simulink subsystem "UAV_model"  (R2025b)
settings: Solver=VariableStepAuto  StartTime=0.0  StopTime=10.0  RelTol=1e-3
values from neighbouring files (symbols this model uses):
  g_noise = 0.01    [random_init.m]
  Ts = 0.05    [generate_commande_preview.m]    (also in random_init.m)
libraries: simulink x18
settings Model: Creator=Max  LastModifiedBy=cs_fondation

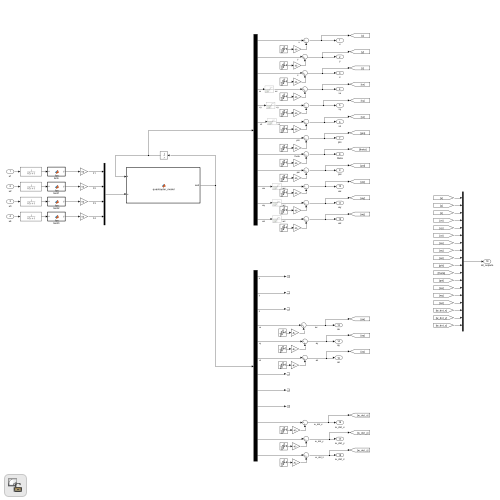
[thumbnail: Simulink's stored preview of the top-level diagram]
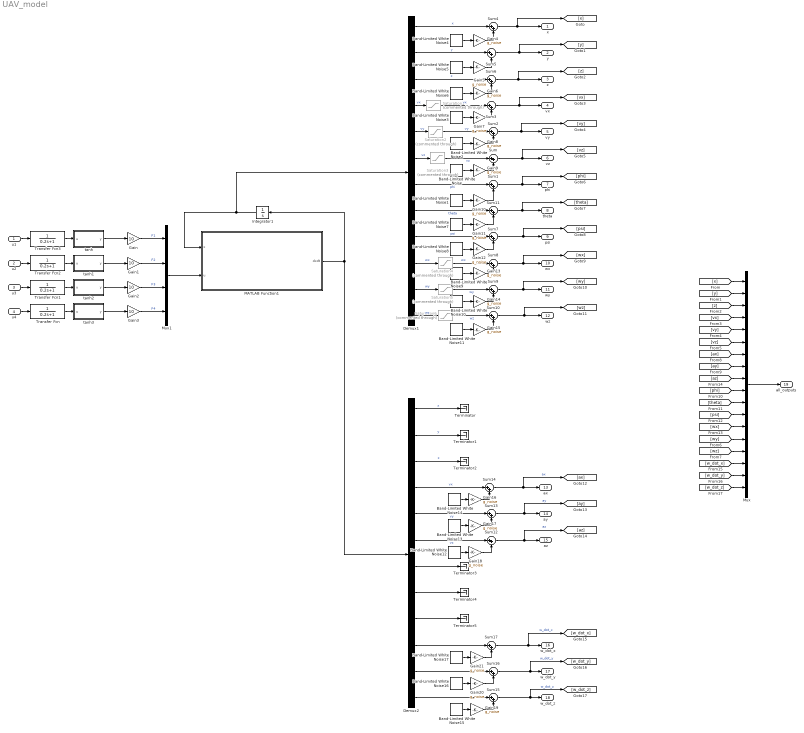
== system UAV_model ==
  u1 : Inport
  u2 : Inport  Port=2
  u3 : Inport  Port=3
  u4 : Inport  Port=4
  Band-Limited White Noise : simulink/Sources/Band-Limited White Noise  Cov=[0.0001]  Ts=Ts  seed=seed_vz
  Band-Limited White Noise1 : simulink/Sources/Band-Limited White Noise  Cov=[0.0001]  Ts=Ts  seed=seed_phi
  Band-Limited White Noise10 : simulink/Sources/Band-Limited White Noise  Cov=[0.0001]  Ts=Ts  seed=seed_wy
  Band-Limited White Noise11 : simulink/Sources/Band-Limited White Noise  Cov=[0.0001]  Ts=Ts  seed=seed_wz
  Band-Limited White Noise12 : simulink/Sources/Band-Limited White Noise  Cov=[0.0001]  Ts=Ts  seed=seed_az
  Band-Limited White Noise13 : simulink/Sources/Band-Limited White Noise  Cov=[0.0001]  Ts=Ts  seed=seed_ay
  Band-Limited White Noise14 : simulink/Sources/Band-Limited White Noise  Cov=[0.0001]  Ts=Ts  seed=seed_ax
  Band-Limited White Noise15 : simulink/Sources/Band-Limited White Noise  Cov=[0.0001]  Ts=Ts  seed=seed_w_dot_z
  Band-Limited White Noise16 : simulink/Sources/Band-Limited White Noise  Cov=[0.0001]  Ts=Ts  seed=seed_w_dot_y
  Band-Limited White Noise17 : simulink/Sources/Band-Limited White Noise  Cov=[0.0001]  Ts=Ts  seed=seed_w_dot_x
  Band-Limited White Noise2 : simulink/Sources/Band-Limited White Noise  Cov=[0.0001]  Ts=Ts  seed=seed_vy
  Band-Limited White Noise3 : simulink/Sources/Band-Limited White Noise  Cov=[0.0001]  Ts=Ts  seed=seed_vx
  Band-Limited White Noise4 : simulink/Sources/Band-Limited White Noise  Cov=[0.0001]  Ts=Ts  seed=seed_x
  Band-Limited White Noise5 : simulink/Sources/Band-Limited White Noise  Cov=[0.0001]  Ts=Ts  seed=seed_y
  Band-Limited White Noise6 : simulink/Sources/Band-Limited White Noise  Cov=[0.0001]  Ts=Ts  seed=seed_z
  Band-Limited White Noise7 : simulink/Sources/Band-Limited White Noise  Cov=[0.0001]  Ts=Ts  seed=[23348]
  Band-Limited White Noise8 : simulink/Sources/Band-Limited White Noise  Cov=[0.0001]  Ts=Ts  seed=seed_psi
  Band-Limited White Noise9 : simulink/Sources/Band-Limited White Noise  Cov=[0.0001]  Ts=Ts  seed=seed_wx
  Demux1 : Demux  Outputs=12
  Demux2 : Demux  Outputs=12
  Gain{,1..3} (4 alike) : Gain  Gain=10
  Gain{4..21} (18 alike) : Gain  Gain=g_noise
  Integrator1 : Integrator  InitialCondition=zeros(12,1)
  MATLAB Function1 : MATLAB Function  TreatAsAtomicUnit=on
  Mux : Mux  Inputs=18
  Mux1 : Mux
  Saturation1 : Saturate  Commented=through  UpperLimit=10  LowerLimit=-10
  Saturation2 : Saturate  Commented=through  UpperLimit=10  LowerLimit=-10
  Saturation3 : Saturate  Commented=through  UpperLimit=10  LowerLimit=-10
  Saturation4 : Saturate  Commented=through  UpperLimit=2  LowerLimit=-2
  Saturation5 : Saturate  Commented=through  UpperLimit=2  LowerLimit=-2
  Saturation6 : Saturate  Commented=through  UpperLimit=2  LowerLimit=-2
  Sum{,1..17} (18 alike) : Sum  Inputs=|++
  Terminator{,1..5} (6 alike) : Terminator
  Transfer Fcn{,1..3} (4 alike) : TransferFcn  Denominator=[0.2 1]
  tanh : MATLAB Function  TreatAsAtomicUnit=on
  tanh1 : MATLAB Function  TreatAsAtomicUnit=on
  tanh2 : MATLAB Function  TreatAsAtomicUnit=on
  tanh3 : MATLAB Function  TreatAsAtomicUnit=on
  x : Outport
  y : Outport  Port=2
  z : Outport  Port=3
  vx : Outport  Port=4
  vy : Outport  Port=5
  vz : Outport  Port=6
  phi : Outport  Port=7
  theta : Outport  Port=8
  psi : Outport  Port=9
  wx : Outport  Port=10
  wy : Outport  Port=11
  wz : Outport  Port=12
  ax : Outport  Port=13
  ay : Outport  Port=14
  az : Outport  Port=15
  w_dot_x : Outport  Port=16
  w_dot_y : Outport  Port=17
  w_dot_z : Outport  Port=18
  all_outputs : Outport  Port=19
  wires:
  Integrator1/1 -> MATLAB Function1/1(x), Demux1/1
  Gain2/1 -> Mux1/3  "F3"
  tanh/1(y) -> Gain/1
  Demux1/1 -> Sum4/1  "x"
  tanh3/1(y) -> Gain3/1
  Demux1/12 -> Saturation6/1  "wz"
  Gain1/1 -> Mux1/2  "F2"
  Gain3/1 -> Mux1/4  "F4"
  MATLAB Function1/1(dxdt) -> Integrator1/1, Demux2/1
  tanh1/1(y) -> Gain1/1
  Gain/1 -> Mux1/1  "F1"
  tanh2/1(y) -> Gain2/1
  Demux1/2 -> Sum5/1  "y"
  Mux1/1 -> MATLAB Function1/2(u)
  Demux1/8 -> Sum11/1  "theta"
  Demux1/11 -> Saturation5/1  "wy"
  Demux1/10 -> Saturation4/1  "wx"
  Demux1/9 -> Sum7/1  "psi"
  Demux1/7 -> Sum1/1  "phi"
  Demux1/4 -> Saturation1/1  "vx"
  u3/1 -> Transfer Fcn1/1
  Demux1/6 -> Saturation3/1  "vz"
  u4/1 -> Transfer Fcn/1
  u2/1 -> Transfer Fcn2/1
  u1/1 -> Transfer Fcn3/1
  Demux1/5 -> Saturation2/1  "vy"
  Transfer Fcn3/1 -> tanh/1(u)
  Transfer Fcn2/1 -> tanh1/1(u)
  Transfer Fcn1/1 -> tanh2/1(u)
  Transfer Fcn/1 -> tanh3/1(u)
  Demux1/3 -> Sum6/1  "z"
  Saturation1/1 -> Sum3/1  "vx"
  Saturation2/1 -> Sum2/1  "vy"
  Saturation3/1 -> Sum/1  "vz"
  Saturation4/1 -> Sum8/1  "wx"
  Saturation5/1 -> Sum9/1  "wy"
  Saturation6/1 -> Sum10/1  "wz"
  Sum/1 -> vz/1, [vz]
  Band-Limited White Noise/1 -> Gain9/1
  Band-Limited White Noise1/1 -> Gain10/1
  Sum1/1 -> phi/1, [phi]
  Band-Limited White Noise2/1 -> Gain8/1
  Sum2/1 -> vy/1, [vy]
  Band-Limited White Noise3/1 -> Gain7/1
  Sum3/1 -> vx/1, [vx]
  Sum4/1 -> x/1, [x]
  Band-Limited White Noise4/1 -> Gain4/1
  Sum5/1 -> y/1, [y]
  Band-Limited White Noise5/1 -> Gain5/1
  Sum6/1 -> z/1, [z]
  Band-Limited White Noise6/1 -> Gain6/1
  Sum11/1 -> theta/1, [theta]
  Sum7/1 -> psi/1, [psi]
  Sum8/1 -> wx/1, [wx]
  Sum9/1 -> wy/1, [wy]
  Band-Limited White Noise7/1 -> Gain11/1
  Band-Limited White Noise8/1 -> Gain12/1
  Band-Limited White Noise9/1 -> Gain13/1
  Band-Limited White Noise10/1 -> Gain14/1
  Band-Limited White Noise11/1 -> Gain15/1
  Sum10/1 -> wz/1, [wz]
  Sum14/1 -> ax/1, [ax]  "ax"
  Sum12/1 -> az/1, [az]  "az"
  Demux2/6 -> Sum12/1  "vz"
  Demux2/5 -> Sum13/1  "vy"
  Demux2/4 -> Sum14/1  "vx"
  Band-Limited White Noise12/1 -> Gain18/1
  Band-Limited White Noise13/1 -> Gain17/1
  Sum13/1 -> ay/1, [ay]  "ay"
  Band-Limited White Noise14/1 -> Gain16/1
  Demux2/3 -> Terminator2/1  "z"
  Demux2/2 -> Terminator1/1  "y"
  Demux2/1 -> Terminator/1  "x"
  Band-Limited White Noise17/1 -> Gain21/1
  Sum16/1 -> w_dot_y/1, [w_dot_y]  "w_dot_y"
  Band-Limited White Noise16/1 -> Gain20/1
  Band-Limited White Noise15/1 -> Gain19/1
  Demux2/10 -> Sum17/1
  Demux2/11 -> Sum16/1
  Demux2/12 -> Sum15/1
  Sum15/1 -> w_dot_z/1, [w_dot_z]  "w_dot_z"
  Sum17/1 -> w_dot_x/1, [w_dot_x]  "w_dot_x"
  Demux2/7 -> Terminator3/1
  Demux2/8 -> Terminator4/1
  Demux2/9 -> Terminator5/1
  [x] -> Mux/1
  [y] -> Mux/2
  [z] -> Mux/3
  [vx] -> Mux/4
  [vy] -> Mux/5
  [vz] -> Mux/6
  [ax] -> Mux/7
  [ay] -> Mux/8
  [az] -> Mux/9
  [phi] -> Mux/10
  [theta] -> Mux/11
  [psi] -> Mux/12
  [wx] -> Mux/13
  [wy] -> Mux/14
  [wz] -> Mux/15
  [w_dot_x] -> Mux/16
  [w_dot_y] -> Mux/17
  [w_dot_z] -> Mux/18
  Mux/1 -> all_outputs/1
  Gain4/1 -> Sum4/2
  Gain5/1 -> Sum5/2
  Gain6/1 -> Sum6/2
  Gain7/1 -> Sum3/2
  Gain8/1 -> Sum2/2
  Gain9/1 -> Sum/2
  Gain10/1 -> Sum1/2
  Gain11/1 -> Sum11/2
  Gain12/1 -> Sum7/2
  Gain13/1 -> Sum8/2
  Gain14/1 -> Sum9/2
  Gain15/1 -> Sum10/2
  Gain16/1 -> Sum14/2
  Gain17/1 -> Sum13/2
  Gain18/1 -> Sum12/2
  Gain19/1 -> Sum15/2
  Gain20/1 -> Sum16/2
  Gain21/1 -> Sum17/2

== matlab function UAV_model/MATLAB Function1 ==
  data: x input; u input; dxdt output
function dxdt = quadcopter_model(x, u)
  
    dxdt = quadcopter_model(x, u);

end

== matlab function UAV_model/tanh1 ==
  data: u input; y output
function y = fcn(u)

    y = tanh(u);

end

== matlab function UAV_model/tanh2 ==
  data: u input; y output
function y = fcn(u)

    y = tanh(u);

end

== matlab function UAV_model/tanh3 ==
  data: u input; y output
function y = fcn(u)

    y = tanh(u);

end

== matlab function UAV_model/tanh ==
  data: u input; y output
function y = fcn(u)

    y = tanh(u);

end
